simulink model "FMS1"  (R2018b)
settings: configuration reference "fms_config" (kept outside this file)
values from neighbouring files (symbols this model uses):
  FMS_EXPORT = Simulink.Parameter(FMS_EXPORT_VALUE)    [fms_model_init.m]
  FMS_PARAM = Simulink.Parameter(FMS_PARAM_VALUE)    [fms_model_init.m]
undefined symbols (not defined in the file or in its folder): actuator_cmd, ax_cmd, ay_cmd, az_cmd, cmd_mask, ControlMode, ctrl_mode, DiscIntNeverNeededParam, FMS_Cmd, FMS_CONST, home, mode, p_cmd, phi_cmd, PilotMode, psi_rate_cmd, q_cmd, r_cmd, reset, state, status, theta_cmd, throttle_cmd, timestamp, u_cmd, v_cmd, VehicleState, VehicleStatus, w_cmd, wp_consume, wp_current
libraries: simulink x119, FMT_Model_Lib x56, hdlsllib x13
(part 6 of 7)

== system FMS1/FMS Commander/Commander/Arm/Auto/Mission/Mission_SubSystem/Velocity Commander/Hold Position/Altitude Hold/Detect Movement ==
  FMS_In : Inport
  Abs : Abs
  Bus Selector : BusSelector  OutputSignals=INS_Out.vd
  Constant : Constant  Value=0  OutDataTypeStr=Inherit: Inherit via back propagation
  Motion Status : Stateflow chart  TreatAsAtomicUnit=on
  motion_state : Outport
  wires:
  FMS_In/1 -> Bus Selector/1
  Motion Status/1(state) -> motion_state/1
  Constant/1 -> Motion Status/1(motion_req)
  Abs/1 -> Motion Status/2(speed)
  Bus Selector/1 -> Abs/1  "<vd>"

== system FMS1/FMS Commander/Commander/Arm/Auto/Mission/Mission_SubSystem/Velocity Commander/Hold Position/Position Hold/Controller ==
  motion_state : Inport
  In Bus Element : Inport  Port=2  PortName=FMS_In
  In Bus Element1 : Inport  Port=2  PortName=FMS_In
  Brake Control : Subsystem  TreatAsAtomicUnit=on
  Hold Control : Subsystem  TreatAsAtomicUnit=on
  Merge : Merge  Inputs=3
  Move Control : Subsystem  TreatAsAtomicUnit=on
  Saturation1 : Saturate  UpperLimit=FMS_PARAM.VEL_XY_LIM  LowerLimit=-FMS_PARAM.VEL_XY_LIM
  Switch Case : SwitchCase  CaseConditions={MotionState.Hold, MotionState.Brake, MotionState.Move}  ShowDefaultCase=off
  uv_cmd_mPs : Outport
  wires:
  Move Control/1(uv_cmd_mPs) -> Merge/3
  Brake Control/1(uv_cmd_mPs) -> Merge/2
  Hold Control/1(uv_cmd_mPs) -> Merge/1
  In Bus Element/1 -> Hold Control/1(FMS_In)
  Switch Case/3 -> Move Control/Action
  Switch Case/2 -> Brake Control/Action
  Switch Case/1 -> Hold Control/Action
  motion_state/1 -> Switch Case/1
  Saturation1/1 -> uv_cmd_mPs/1
  Merge/1 -> Saturation1/1
  In Bus Element1/1 -> Move Control/1(FMS_In)

== system FMS1/FMS Commander/Commander/Arm/Auto/Mission/Mission_SubSystem/Velocity Commander/Hold Position/Position Hold/Detect Movement ==
  FMS_In : Inport
  Add : Sum
  Bus Selector1 : BusSelector  OutputSignals=INS_Out.vn,INS_Out.ve
  Constant : Constant  Value=0  OutDataTypeStr=Inherit: Inherit via back propagation
  Motion State : Stateflow chart  TreatAsAtomicUnit=on
  Sqrt : Sqrt  SaturateOnIntegerOverflow=on
  Square : Math  Operator=square  SaturateOnIntegerOverflow=on
  Square1 : Math  Operator=square  SaturateOnIntegerOverflow=on
  motion_state : Outport
  wires:
  FMS_In/1 -> Bus Selector1/1
  Add/1 -> Sqrt/1
  Square1/1 -> Add/2
  Square/1 -> Add/1
  Motion State/1(state) -> motion_state/1  "pos_ms"
  Sqrt/1 -> Motion State/2(speed)
  Bus Selector1/1 -> Square/1  "<vn>"
  Bus Selector1/2 -> Square1/1  "<ve>"
  Constant/1 -> Motion State/1(motion_req)

== system FMS1/FMS Commander/Commander/Arm/SubMode/Hold/Altitude Hold/Controller/Move Control/TD1/fhan  ==
  v1 : Inport
  v2 : Inport  Port=2
  Abs : Abs
  Add{,1..3,5..6} (6 alike) : Sum  OutDataTypeStr=Inherit: Same as first input
  Add4 : Sum  Inputs=-++
  Divide : Product  Inputs=*/
  Gain : Gain  Gain=8
  Gain1 : Gain  Gain=0.5  OutDataTypeStr=Inherit: Same as input
  Gain2 : Gain  Gain=0.5  OutDataTypeStr=Inherit: Same as input
  Gain3 : Gain  Gain=0.5  OutDataTypeStr=Inherit: Same as input
  Gain4 : Gain  Gain=-1  OutDataTypeStr=Inherit: Same as input
  Multiply{,1..3} (4 alike) : Product  OutDataTypeStr=Inherit: Same as first input
  Multiply4 : Product  OutDataTypeStr=single
  Multiply5 : Product  Inputs=3
  Multiply6 : Product  OutDataTypeStr=single
  Sign{,1..6} (7 alike) : Signum
  Sqrt : Sqrt  SaturateOnIntegerOverflow=on
  Square : Math  Operator=square  SaturateOnIntegerOverflow=on
  Subtract{,1..5} (6 alike) : Sum  Inputs=+-  OutDataTypeStr=Inherit: Same as first input
  Subtract6 : Sum  Inputs=-+  OutDataTypeStr=Inherit: Same as first input
  const : Constant  Value=r0  OutDataTypeStr=single
  const1 : Constant  Value=h0  OutDataTypeStr=single
  fhan : Outport
  wires:
  Sign1/1 -> Subtract2/1
  Multiply2/1 -> Sqrt/1
  Square/1 -> Multiply/2
  Gain1/1 -> Multiply3/2
  Multiply6/1 -> Subtract6/1
  Multiply/1 -> Multiply2/2, Add1/1, Add3/2, Subtract1/2, Add6/2, Subtract3/2, Divide/2, Subtract/2  "d"
  Add6/1 -> Sign3/1
  Sign3/1 -> Subtract4/1
  Sign6/1 -> Multiply6/1
  Multiply5/1 -> Subtract6/2
  Gain4/1 -> Multiply5/1
  Subtract4/1 -> Gain3/1
  Add2/1 -> Add5/1, Add4/1  "a2"
  Subtract2/1 -> Gain2/1
  Add/1 -> Abs/1, Sign/1, Add4/2, Add3/1, Subtract1/1  "y"
  Multiply1/1 -> Add/2, Add2/2, Add4/3  "a0"
  Add5/1 -> Add6/1, Subtract3/1, Divide/1, Sign5/1, Sign6/1  "a"
  const1/1 -> Square/1, Multiply1/2
  Multiply4/1 -> Add5/2
  Subtract5/1 -> Multiply5/2
  Add3/1 -> Sign1/1
  const/1 -> Multiply/1, Gain4/1, Multiply6/2
  Gain/1 -> Add1/2
  Multiply3/1 -> Add2/1
  Divide/1 -> Subtract5/1
  Subtract1/1 -> Sign2/1
  Add1/1 -> Multiply2/1
  Subtract3/1 -> Sign4/1
  Sqrt/1 -> Subtract/1  "a1"
  Sign5/1 -> Subtract5/2
  Add4/1 -> Multiply4/1
  Abs/1 -> Gain/1
  Sign4/1 -> Subtract4/2
  Sign2/1 -> Subtract2/2
  Subtract6/1 -> fhan/1
  Subtract/1 -> Gain1/1
  Gain3/1 -> Multiply5/3  "sa"
  v2/1 -> Multiply1/1
  Gain2/1 -> Multiply4/2  "sy"
  Sign/1 -> Multiply3/1
  v1/1 -> Add/1

== system FMS1/FMS Commander/Commander/Arm/SubMode/Hold/Heading Hold/Controller/Move Control/TD/fhan  ==
  v1 : Inport
  v2 : Inport  Port=2
  Abs : Abs
  Add{,1..3,5..6} (6 alike) : Sum  OutDataTypeStr=Inherit: Same as first input
  Add4 : Sum  Inputs=-++
  Divide : Product  Inputs=*/
  Gain : Gain  Gain=8
  Gain1 : Gain  Gain=0.5  OutDataTypeStr=Inherit: Same as input
  Gain2 : Gain  Gain=0.5  OutDataTypeStr=Inherit: Same as input
  Gain3 : Gain  Gain=0.5  OutDataTypeStr=Inherit: Same as input
  Gain4 : Gain  Gain=-1  OutDataTypeStr=Inherit: Same as input
  Multiply{,1..3} (4 alike) : Product  OutDataTypeStr=Inherit: Same as first input
  Multiply4 : Product  OutDataTypeStr=single
  Multiply5 : Product  Inputs=3
  Multiply6 : Product  OutDataTypeStr=single
  Sign{,1..6} (7 alike) : Signum
  Sqrt : Sqrt  SaturateOnIntegerOverflow=on
  Square : Math  Operator=square  SaturateOnIntegerOverflow=on
  Subtract{,1..5} (6 alike) : Sum  Inputs=+-  OutDataTypeStr=Inherit: Same as first input
  Subtract6 : Sum  Inputs=-+  OutDataTypeStr=Inherit: Same as first input
  const : Constant  Value=r0  OutDataTypeStr=single
  const1 : Constant  Value=h0  OutDataTypeStr=single
  fhan : Outport
  wires:
  v1/1 -> Add/1
  Sign/1 -> Multiply3/1
  Gain2/1 -> Multiply4/2  "sy"
  v2/1 -> Multiply1/1
  Gain3/1 -> Multiply5/3  "sa"
  Subtract/1 -> Gain1/1
  Subtract6/1 -> fhan/1
  Sign2/1 -> Subtract2/2
  Sign4/1 -> Subtract4/2
  Abs/1 -> Gain/1
  Add4/1 -> Multiply4/1
  Sign5/1 -> Subtract5/2
  Sqrt/1 -> Subtract/1  "a1"
  Subtract3/1 -> Sign4/1
  Add1/1 -> Multiply2/1
  Subtract1/1 -> Sign2/1
  Divide/1 -> Subtract5/1
  Multiply3/1 -> Add2/1
  Gain/1 -> Add1/2
  const/1 -> Multiply6/2, Gain4/1, Multiply/1
  Add3/1 -> Sign1/1
  Subtract5/1 -> Multiply5/2
  Multiply4/1 -> Add5/2
  const1/1 -> Multiply1/2, Square/1
  Add5/1 -> Sign6/1, Sign5/1, Divide/1, Subtract3/1, Add6/1  "a"
  Multiply1/1 -> Add4/3, Add2/2, Add/2  "a0"
  Add/1 -> Subtract1/1, Add3/1, Add4/2, Sign/1, Abs/1  "y"
  Subtract2/1 -> Gain2/1
  Add2/1 -> Add4/1, Add5/1  "a2"
  Subtract4/1 -> Gain3/1
  Gain4/1 -> Multiply5/1
  Multiply5/1 -> Subtract6/2
  Sign6/1 -> Multiply6/1
  Sign3/1 -> Subtract4/1
  Add6/1 -> Sign3/1
  Multiply/1 -> Subtract/2, Divide/2, Subtract3/2, Add6/2, Subtract1/2, Add3/2, Add1/1, Multiply2/2  "d"
  Multiply6/1 -> Subtract6/1
  Gain1/1 -> Multiply3/2
  Square/1 -> Multiply/2
  Multiply2/1 -> Sqrt/1
  Sign1/1 -> Subtract2/1

== system FMS1/FMS Commander/Commander/Arm/SubMode/Hold/Position Hold/Controller/Move Control/TD/fhan  ==
  v1 : Inport
  v2 : Inport  Port=2
  Abs : Abs
  Add{,1..3,5..6} (6 alike) : Sum  OutDataTypeStr=Inherit: Same as first input
  Add4 : Sum  Inputs=-++
  Divide : Product  Inputs=*/
  Gain : Gain  Gain=8
  Gain1 : Gain  Gain=0.5  OutDataTypeStr=Inherit: Same as input
  Gain2 : Gain  Gain=0.5  OutDataTypeStr=Inherit: Same as input
  Gain3 : Gain  Gain=0.5  OutDataTypeStr=Inherit: Same as input
  Gain4 : Gain  Gain=-1  OutDataTypeStr=Inherit: Same as input
  Multiply{,1..3} (4 alike) : Product  OutDataTypeStr=Inherit: Same as first input
  Multiply4 : Product  OutDataTypeStr=single
  Multiply5 : Product  Inputs=3
  Multiply6 : Product  OutDataTypeStr=single
  Sign{,1..6} (7 alike) : Signum
  Sqrt : Sqrt  SaturateOnIntegerOverflow=on
  Square : Math  Operator=square  SaturateOnIntegerOverflow=on
  Subtract{,1..5} (6 alike) : Sum  Inputs=+-  OutDataTypeStr=Inherit: Same as first input
  Subtract6 : Sum  Inputs=-+  OutDataTypeStr=Inherit: Same as first input
  const : Constant  Value=r0  OutDataTypeStr=single
  const1 : Constant  Value=h0  OutDataTypeStr=single
  fhan : Outport
  wires:
  v1/1 -> Add/1
  Sign/1 -> Multiply3/1
  Gain2/1 -> Multiply4/2  "sy"
  v2/1 -> Multiply1/1
  Gain3/1 -> Multiply5/3  "sa"
  Subtract/1 -> Gain1/1
  Subtract6/1 -> fhan/1
  Sign2/1 -> Subtract2/2
  Sign4/1 -> Subtract4/2
  Abs/1 -> Gain/1
  Add4/1 -> Multiply4/1
  Sign5/1 -> Subtract5/2
  Sqrt/1 -> Subtract/1  "a1"
  Subtract3/1 -> Sign4/1
  Add1/1 -> Multiply2/1
  Subtract1/1 -> Sign2/1
  Divide/1 -> Subtract5/1
  Multiply3/1 -> Add2/1
  Gain/1 -> Add1/2
  const/1 -> Multiply6/2, Gain4/1, Multiply/1
  Add3/1 -> Sign1/1
  Subtract5/1 -> Multiply5/2
  Multiply4/1 -> Add5/2
  const1/1 -> Multiply1/2, Square/1
  Add5/1 -> Sign6/1, Sign5/1, Divide/1, Subtract3/1, Add6/1  "a"
  Multiply1/1 -> Add4/3, Add2/2, Add/2  "a0"
  Add/1 -> Subtract1/1, Add3/1, Add4/2, Sign/1, Abs/1  "y"
  Subtract2/1 -> Gain2/1
  Add2/1 -> Add4/1, Add5/1  "a2"
  Subtract4/1 -> Gain3/1
  Gain4/1 -> Multiply5/1
  Multiply5/1 -> Subtract6/2
  Sign6/1 -> Multiply6/1
  Sign3/1 -> Subtract4/1
  Add6/1 -> Sign3/1
  Multiply/1 -> Subtract/2, Divide/2, Subtract3/2, Add6/2, Subtract1/2, Add3/2, Add1/1, Multiply2/2  "d"
  Multiply6/1 -> Subtract6/1
  Gain1/1 -> Multiply3/2
  Square/1 -> Multiply/2
  Multiply2/1 -> Sqrt/1
  Sign1/1 -> Subtract2/1

== system FMS1/FMS Commander/Commander/Arm/SubMode/Return/Velocity Commander1/Hold Position/Altitude Hold/Controller/Brake Control ==
  Action Port : ActionPort  InitializeStates=reset  ActionType=case
  Brake Speed : Constant  Value=0  VectorParams1D=off  OutDataTypeStr=single
  psi_rate_cmd_radPs : Outport
  wires:
  Brake Speed/1 -> psi_rate_cmd_radPs/1

== system FMS1/FMS Commander/Commander/Arm/SubMode/Return/Velocity Commander1/Hold Position/Altitude Hold/Controller/Hold Control ==
  FMS_In : Inport
  Action Port : ActionPort  InitializeStates=reset  ActionType=case
  Bus_Selection : Subsystem
  Delay : Delay  DelayLength=1  InitialConditionSource=Input port
      settings: InputPortMap=u0,p4
  Gain2 : Gain  Gain=FMS_PARAM.Z_P  OutDataTypeStr=single
  Sum : Sum  Inputs=-+|
  w_cmd_mPs : Outport
  wires:
  FMS_In/1 -> Bus_Selection/1(FMS_In)
  Delay/1 -> Sum/2, Delay/1  "z_cmd_R"
  Sum/1 -> Gain2/1  "z_err_R"
  Bus_Selection/1(z_R_m) -> Delay/2, Sum/1  "z_est_R"
  Gain2/1 -> w_cmd_mPs/1

== system FMS1/FMS Commander/Commander/Arm/SubMode/Return/Velocity Commander1/Hold Position/Altitude Hold/Controller/Move Control ==
  FMS_In : Inport
  Action Port : ActionPort  InitializeStates=reset  ActionType=case
  Bus Selector : BusSelector  OutputSignals=Pilot_Cmd.stick_throttle
  DeadZone : Subsystem  mask{th=FMS_PARAM.THROTTLE_DZ}
      mask prompts: th "Threshold"
      mask Display: disp('Dead Zone')
  Gain1 : Gain  Gain=-FMS_PARAM.VEL_Z_LIM  OutDataTypeStr=single
  TD1 : Subsystem
  w_cmd_mPs : Outport
  wires:
  TD1/1(v1) -> w_cmd_mPs/1
  FMS_In/1 -> Bus Selector/1
  Bus Selector/1 -> DeadZone/1(u)  "<stick_throttle>"
  DeadZone/1(y) -> Gain1/1
  Gain1/1 -> TD1/1(v)

== system FMS1/FMS Commander/Commander/Arm/SubMode/Return/Velocity Commander1/Hold Position/Position Hold/Controller/Brake Control ==
  Action Port : ActionPort  InitializeStates=reset  ActionType=case
  Brake Speed : Constant  Value=[0;0]  VectorParams1D=off  OutDataTypeStr=single
  uv_cmd_mPs : Outport
  wires:
  Brake Speed/1 -> uv_cmd_mPs/1

== system FMS1/FMS Commander/Commander/Arm/SubMode/Return/Velocity Commander1/Hold Position/Position Hold/Controller/Hold Control ==
  FMS_In : Inport
  Action Port : ActionPort  InitializeStates=reset  ActionType=case
  Bus Selector : BusSelector  OutputSignals=INS_Out.psi
  Bus_Selection : Subsystem
  Constant : Constant  Value=0  OutDataTypeStr=Inherit: Inherit via back propagation
  Delay : Delay  DelayLength=1  InitialConditionSource=Input port
      settings: InputPortMap=u0,p4
  Gain2 : Gain  Gain=FMS_PARAM.XY_P  OutDataTypeStr=single
  Multiply : Product  Multiplication=Matrix(*)
  Mux : Mux  Inputs=2
  Psi To DCM : FMT_Model_Lib/Transformation/Psi To DCM
      settings: SourceProductName=FMT Toolbox
  Selector : Selector  InputPortWidth=3  IndexOptions=Index vector (dialog)  Indices=[1 2]  OutputSizes=1
  Sum : Sum  Inputs=-+|
  uv_cmd_mPs : Outport
  wires:
  Bus Selector/1 -> Psi To DCM/1  "<psi>"
  Selector/1 -> Gain2/1
  Mux/1 -> Multiply/2
  Multiply/1 -> Selector/1
  Psi To DCM/1 -> Multiply/1  "M_CO"
  Constant/1 -> Mux/2
  FMS_In/1 -> Bus_Selection/1(FMS_In), Bus Selector/1
  Delay/1 -> Sum/2, Delay/1  "xy_cmd_R"
  Sum/1 -> Mux/1  "xy_err_R"
  Bus_Selection/1(xy_R_O_m) -> Delay/2, Sum/1  "xy_est_R"
  Gain2/1 -> uv_cmd_mPs/1

== system FMS1/FMS Commander/Commander/Arm/SubMode/Return/Velocity Commander1/Hold Position/Position Hold/Controller/Move Control ==
  FMS_In : Inport
  Action Port : ActionPort  InitializeStates=reset  ActionType=case
  Bus Selector : BusSelector  OutputSignals=Pilot_Cmd.stick_pitch,Pilot_Cmd.stick_roll
  DeadZone : Subsystem  mask{th=FMS_PARAM.PITCH_DZ}
      mask prompts: th "Threshold"
      mask Display: disp('Dead Zone')
  DeadZone1 : Subsystem  mask{th=FMS_PARAM.ROLL_DZ}
      mask prompts: th "Threshold"
      mask Display: disp('Dead Zone')
  Gain6 : Gain  Gain=FMS_PARAM.VEL_XY_LIM  OutDataTypeStr=single
  Mux1 : Mux  Inputs=2
  TD : Subsystem
  uv_cmd_mPs : Outport
  wires:
  Mux1/1 -> Gain6/1
  DeadZone1/1(y) -> Mux1/2
  Bus Selector/2 -> DeadZone1/1(u)  "<stick_roll>"
  TD/1(v1) -> uv_cmd_mPs/1
  FMS_In/1 -> Bus Selector/1
  Bus Selector/1 -> DeadZone/1(u)  "<stick_pitch>"
  DeadZone/1(y) -> Mux1/1
  Gain6/1 -> TD/1(v)

== system FMS1/FMS Commander/Commander/Arm/Auto/Mission/Mission_SubSystem/Velocity Commander/Hold Position/Altitude Hold/Controller/Brake Control ==
  Action Port : ActionPort  InitializeStates=reset  ActionType=case
  Brake Speed : Constant  Value=0  VectorParams1D=off  OutDataTypeStr=single
  psi_rate_cmd_radPs : Outport
  wires:
  Brake Speed/1 -> psi_rate_cmd_radPs/1

== system FMS1/FMS Commander/Commander/Arm/Auto/Mission/Mission_SubSystem/Velocity Commander/Hold Position/Altitude Hold/Controller/Hold Control ==
  FMS_In : Inport
  Action Port : ActionPort  InitializeStates=reset  ActionType=case
  Bus_Selection : Subsystem
  Delay : Delay  DelayLength=1  InitialConditionSource=Input port
      settings: InputPortMap=u0,p4
  Gain2 : Gain  Gain=FMS_PARAM.Z_P  OutDataTypeStr=single
  Sum : Sum  Inputs=-+|
  w_cmd_mPs : Outport
  wires:
  FMS_In/1 -> Bus_Selection/1(FMS_In)
  Delay/1 -> Sum/2, Delay/1  "z_cmd_R"
  Sum/1 -> Gain2/1  "z_err_R"
  Bus_Selection/1(z_R_m) -> Delay/2, Sum/1  "z_est_R"
  Gain2/1 -> w_cmd_mPs/1

== system FMS1/FMS Commander/Commander/Arm/Auto/Mission/Mission_SubSystem/Velocity Commander/Hold Position/Altitude Hold/Controller/Move Control ==
  FMS_In : Inport
  Action Port : ActionPort  InitializeStates=reset  ActionType=case
  Bus Selector : BusSelector  OutputSignals=Pilot_Cmd.stick_throttle
  DeadZone : Subsystem  mask{th=FMS_PARAM.THROTTLE_DZ}
      mask prompts: th "Threshold"
      mask Display: disp('Dead Zone')
  Gain1 : Gain  Gain=-FMS_PARAM.VEL_Z_LIM  OutDataTypeStr=single
  TD1 : Subsystem
  w_cmd_mPs : Outport
  wires:
  TD1/1(v1) -> w_cmd_mPs/1
  FMS_In/1 -> Bus Selector/1
  Bus Selector/1 -> DeadZone/1(u)  "<stick_throttle>"
  DeadZone/1(y) -> Gain1/1
  Gain1/1 -> TD1/1(v)

== system FMS1/FMS Commander/Commander/Arm/Auto/Mission/Mission_SubSystem/Velocity Commander/Hold Position/Position Hold/Controller/Brake Control ==
  Action Port : ActionPort  InitializeStates=reset  ActionType=case
  Brake Speed : Constant  Value=[0;0]  VectorParams1D=off  OutDataTypeStr=single
  uv_cmd_mPs : Outport
  wires:
  Brake Speed/1 -> uv_cmd_mPs/1

== system FMS1/FMS Commander/Commander/Arm/Auto/Mission/Mission_SubSystem/Velocity Commander/Hold Position/Position Hold/Controller/Hold Control ==
  FMS_In : Inport
  Action Port : ActionPort  InitializeStates=reset  ActionType=case
  Bus Selector : BusSelector  OutputSignals=INS_Out.psi
  Bus_Selection : Subsystem
  Constant : Constant  Value=0  OutDataTypeStr=Inherit: Inherit via back propagation
  Delay : Delay  DelayLength=1  InitialConditionSource=Input port
      settings: InputPortMap=u0,p4
  Gain2 : Gain  Gain=FMS_PARAM.XY_P  OutDataTypeStr=single
  Multiply : Product  Multiplication=Matrix(*)
  Mux : Mux  Inputs=2
  Psi To DCM : FMT_Model_Lib/Transformation/Psi To DCM
      settings: SourceProductName=FMT Toolbox
  Selector : Selector  InputPortWidth=3  IndexOptions=Index vector (dialog)  Indices=[1 2]  OutputSizes=1
  Sum : Sum  Inputs=-+|
  uv_cmd_mPs : Outport
  wires:
  Bus Selector/1 -> Psi To DCM/1  "<psi>"
  Selector/1 -> Gain2/1
  Mux/1 -> Multiply/2
  Multiply/1 -> Selector/1
  Psi To DCM/1 -> Multiply/1  "M_CO"
  Constant/1 -> Mux/2
  FMS_In/1 -> Bus_Selection/1(FMS_In), Bus Selector/1
  Delay/1 -> Sum/2, Delay/1  "xy_cmd_R"
  Sum/1 -> Mux/1  "xy_err_R"
  Bus_Selection/1(xy_R_O_m) -> Delay/2, Sum/1  "xy_est_R"
  Gain2/1 -> uv_cmd_mPs/1

== system FMS1/FMS Commander/Commander/Arm/Auto/Mission/Mission_SubSystem/Velocity Commander/Hold Position/Position Hold/Controller/Move Control ==
  FMS_In : Inport
  Action Port : ActionPort  InitializeStates=reset  ActionType=case
  Bus Selector : BusSelector  OutputSignals=Pilot_Cmd.stick_pitch,Pilot_Cmd.stick_roll
  DeadZone : Subsystem  mask{th=FMS_PARAM.PITCH_DZ}
      mask prompts: th "Threshold"
      mask Display: disp('Dead Zone')
  DeadZone1 : Subsystem  mask{th=FMS_PARAM.ROLL_DZ}
      mask prompts: th "Threshold"
      mask Display: disp('Dead Zone')
  Gain6 : Gain  Gain=FMS_PARAM.VEL_XY_LIM  OutDataTypeStr=single
  Mux1 : Mux  Inputs=2
  TD : Subsystem
  uv_cmd_mPs : Outport
  wires:
  Mux1/1 -> Gain6/1
  DeadZone1/1(y) -> Mux1/2
  Bus Selector/2 -> DeadZone1/1(u)  "<stick_roll>"
  TD/1(v1) -> uv_cmd_mPs/1
  FMS_In/1 -> Bus Selector/1
  Bus Selector/1 -> DeadZone/1(u)  "<stick_pitch>"
  DeadZone/1(y) -> Mux1/1
  Gain6/1 -> TD/1(v)

== system FMS1/FMS Commander/Commander/Arm/SubMode/Return/Velocity Commander1/Hold Position/Altitude Hold/Controller/Hold Control/Bus_Selection ==
  FMS_In : Inport
  Bus Selector2 : BusSelector  OutputSignals=INS_Out.h_R
  Gain : Gain  Gain=-1
  z_R_m : Outport
  wires:
  Gain/1 -> z_R_m/1
  Bus Selector2/1 -> Gain/1  "<h_R>"
  FMS_In/1 -> Bus Selector2/1

== system FMS1/FMS Commander/Commander/Arm/SubMode/Return/Velocity Commander1/Hold Position/Altitude Hold/Controller/Move Control/DeadZone ==
  u : Inport
  Dead Zone : DeadZone  LowerValue=-th  UpperValue=th  SaturateOnIntegerOverflow=on
  Gain : Gain  Gain=1/(1-th)
  y : Outport
  wires:
  Gain/1 -> y/1
  Dead Zone/1 -> Gain/1
  u/1 -> Dead Zone/1

== system FMS1/FMS Commander/Commander/Arm/SubMode/Return/Velocity Commander1/Hold Position/Altitude Hold/Controller/Move Control/TD1 ==
  v : Inport
  Integrator : DiscreteIntegrator  SampleTime=-1  ICPrevOutput=DiscIntNeverNeededParam  ICPrevScaledInput=DiscIntNeverNeededParam
  Integrator1 : DiscreteIntegrator  SampleTime=-1  ICPrevOutput=DiscIntNeverNeededParam  ICPrevScaledInput=DiscIntNeverNeededParam
  Subtract : Sum  Inputs=+-
  "fhan " : Subsystem  mask{r0=8*9.806, h0=0.05}
      mask DialogControl ParameterGroupVar Prompt: fhan(v1,v2,r0,h0)
  v1 : Outport
  wires:
  Integrator1/1 -> v1/1, Subtract/1
  v/1 -> Subtract/2
  Integrator/1 -> "fhan "/2(v2), Integrator1/1  "v2"
  Subtract/1 -> "fhan "/1(v1)
  "fhan "/1(fhan) -> Integrator/1

== system FMS1/FMS Commander/Commander/Arm/SubMode/Return/Velocity Commander1/Hold Position/Position Hold/Controller/Hold Control/Bus_Selection ==
  FMS_In : Inport
  Bus Selector2 : BusSelector  OutputSignals=INS_Out.x_R,INS_Out.y_R
  Mux : Mux  Inputs=2
  xy_R_O_m : Outport
  wires:
  Bus Selector2/2 -> Mux/2  "<y_R>"
  Mux/1 -> xy_R_O_m/1
  Bus Selector2/1 -> Mux/1  "<x_R>"
  FMS_In/1 -> Bus Selector2/1

== system FMS1/FMS Commander/Commander/Arm/SubMode/Return/Velocity Commander1/Hold Position/Position Hold/Controller/Move Control/DeadZone ==
  u : Inport
  Dead Zone : DeadZone  LowerValue=-th  UpperValue=th  SaturateOnIntegerOverflow=on
  Gain : Gain  Gain=1/(1-th)
  y : Outport
  wires:
  Gain/1 -> y/1
  Dead Zone/1 -> Gain/1
  u/1 -> Dead Zone/1

== system FMS1/FMS Commander/Commander/Arm/SubMode/Return/Velocity Commander1/Hold Position/Position Hold/Controller/Move Control/DeadZone1 ==
  u : Inport
  Dead Zone : DeadZone  LowerValue=-th  UpperValue=th  SaturateOnIntegerOverflow=on
  Gain : Gain  Gain=1/(1-th)
  y : Outport
  wires:
  u/1 -> Dead Zone/1
  Dead Zone/1 -> Gain/1
  Gain/1 -> y/1

== system FMS1/FMS Commander/Commander/Arm/SubMode/Return/Velocity Commander1/Hold Position/Position Hold/Controller/Move Control/TD ==
  v : Inport
  Integrator : DiscreteIntegrator  SampleTime=-1  ICPrevOutput=DiscIntNeverNeededParam  ICPrevScaledInput=DiscIntNeverNeededParam
  Integrator1 : DiscreteIntegrator  SampleTime=-1  ICPrevOutput=DiscIntNeverNeededParam  ICPrevScaledInput=DiscIntNeverNeededParam
  Subtract : Sum  Inputs=+-
  "fhan " : Subsystem  mask{r0=6*9.806, h0=0.05}
      mask DialogControl ParameterGroupVar Prompt: fhan(v1,v2,r0,h0)
  v1 : Outport
  wires:
  "fhan "/1(fhan) -> Integrator/1
  Subtract/1 -> "fhan "/1(v1)
  Integrator/1 -> Integrator1/1, "fhan "/2(v2)  "v2"
  v/1 -> Subtract/2
  Integrator1/1 -> Subtract/1, v1/1

== system FMS1/FMS Commander/Commander/Arm/Auto/Mission/Mission_SubSystem/Velocity Commander/Hold Position/Altitude Hold/Controller/Hold Control/Bus_Selection ==
  FMS_In : Inport
  Bus Selector2 : BusSelector  OutputSignals=INS_Out.h_R
  Gain : Gain  Gain=-1
  z_R_m : Outport
  wires:
  Gain/1 -> z_R_m/1
  Bus Selector2/1 -> Gain/1  "<h_R>"
  FMS_In/1 -> Bus Selector2/1

== system FMS1/FMS Commander/Commander/Arm/Auto/Mission/Mission_SubSystem/Velocity Commander/Hold Position/Altitude Hold/Controller/Move Control/DeadZone ==
  u : Inport
  Dead Zone : DeadZone  LowerValue=-th  UpperValue=th  SaturateOnIntegerOverflow=on
  Gain : Gain  Gain=1/(1-th)
  y : Outport
  wires:
  Gain/1 -> y/1
  Dead Zone/1 -> Gain/1
  u/1 -> Dead Zone/1

== system FMS1/FMS Commander/Commander/Arm/Auto/Mission/Mission_SubSystem/Velocity Commander/Hold Position/Altitude Hold/Controller/Move Control/TD1 ==
  v : Inport
  Integrator : DiscreteIntegrator  SampleTime=-1  ICPrevOutput=DiscIntNeverNeededParam  ICPrevScaledInput=DiscIntNeverNeededParam
  Integrator1 : DiscreteIntegrator  SampleTime=-1  ICPrevOutput=DiscIntNeverNeededParam  ICPrevScaledInput=DiscIntNeverNeededParam
  Subtract : Sum  Inputs=+-
  "fhan " : Subsystem  mask{r0=8*9.806, h0=0.05}
      mask DialogControl ParameterGroupVar Prompt: fhan(v1,v2,r0,h0)
  v1 : Outport
  wires:
  Integrator1/1 -> v1/1, Subtract/1
  v/1 -> Subtract/2
  Integrator/1 -> "fhan "/2(v2), Integrator1/1  "v2"
  Subtract/1 -> "fhan "/1(v1)
  "fhan "/1(fhan) -> Integrator/1

== system FMS1/FMS Commander/Commander/Arm/Auto/Mission/Mission_SubSystem/Velocity Commander/Hold Position/Position Hold/Controller/Hold Control/Bus_Selection ==
  FMS_In : Inport
  Bus Selector2 : BusSelector  OutputSignals=INS_Out.x_R,INS_Out.y_R
  Mux : Mux  Inputs=2
  xy_R_O_m : Outport
  wires:
  Bus Selector2/2 -> Mux/2  "<y_R>"
  Mux/1 -> xy_R_O_m/1
  Bus Selector2/1 -> Mux/1  "<x_R>"
  FMS_In/1 -> Bus Selector2/1

== system FMS1/FMS Commander/Commander/Arm/Auto/Mission/Mission_SubSystem/Velocity Commander/Hold Position/Position Hold/Controller/Move Control/DeadZone ==
  u : Inport
  Dead Zone : DeadZone  LowerValue=-th  UpperValue=th  SaturateOnIntegerOverflow=on
  Gain : Gain  Gain=1/(1-th)
  y : Outport
  wires:
  Gain/1 -> y/1
  Dead Zone/1 -> Gain/1
  u/1 -> Dead Zone/1

== system FMS1/FMS Commander/Commander/Arm/Auto/Mission/Mission_SubSystem/Velocity Commander/Hold Position/Position Hold/Controller/Move Control/DeadZone1 ==
  u : Inport
  Dead Zone : DeadZone  LowerValue=-th  UpperValue=th  SaturateOnIntegerOverflow=on
  Gain : Gain  Gain=1/(1-th)
  y : Outport
  wires:
  u/1 -> Dead Zone/1
  Dead Zone/1 -> Gain/1
  Gain/1 -> y/1

== system FMS1/FMS Commander/Commander/Arm/Auto/Mission/Mission_SubSystem/Velocity Commander/Hold Position/Position Hold/Controller/Move Control/TD ==
  v : Inport
  Integrator : DiscreteIntegrator  SampleTime=-1  ICPrevOutput=DiscIntNeverNeededParam  ICPrevScaledInput=DiscIntNeverNeededParam
  Integrator1 : DiscreteIntegrator  SampleTime=-1  ICPrevOutput=DiscIntNeverNeededParam  ICPrevScaledInput=DiscIntNeverNeededParam
  Subtract : Sum  Inputs=+-
  "fhan " : Subsystem  mask{r0=6*9.806, h0=0.05}
      mask DialogControl ParameterGroupVar Prompt: fhan(v1,v2,r0,h0)
  v1 : Outport
  wires:
  "fhan "/1(fhan) -> Integrator/1
  Subtract/1 -> "fhan "/1(v1)
  Integrator/1 -> Integrator1/1, "fhan "/2(v2)  "v2"
  v/1 -> Subtract/2
  Integrator1/1 -> Subtract/1, v1/1

== system FMS1/FMS Commander/Commander/Arm/SubMode/Return/Velocity Commander1/Hold Position/Altitude Hold/Controller/Move Control/TD1/fhan  ==
  v1 : Inport
  v2 : Inport  Port=2
  Abs : Abs
  Add{,1..3,5..6} (6 alike) : Sum  OutDataTypeStr=Inherit: Same as first input
  Add4 : Sum  Inputs=-++
  Divide : Product  Inputs=*/
  Gain : Gain  Gain=8
  Gain1 : Gain  Gain=0.5  OutDataTypeStr=Inherit: Same as input
  Gain2 : Gain  Gain=0.5  OutDataTypeStr=Inherit: Same as input
  Gain3 : Gain  Gain=0.5  OutDataTypeStr=Inherit: Same as input
  Gain4 : Gain  Gain=-1  OutDataTypeStr=Inherit: Same as input
  Multiply{,1..3} (4 alike) : Product  OutDataTypeStr=Inherit: Same as first input
  Multiply4 : Product  OutDataTypeStr=single
  Multiply5 : Product  Inputs=3
  Multiply6 : Product  OutDataTypeStr=single
  Sign{,1..6} (7 alike) : Signum
  Sqrt : Sqrt  SaturateOnIntegerOverflow=on
  Square : Math  Operator=square  SaturateOnIntegerOverflow=on
  Subtract{,1..5} (6 alike) : Sum  Inputs=+-  OutDataTypeStr=Inherit: Same as first input
  Subtract6 : Sum  Inputs=-+  OutDataTypeStr=Inherit: Same as first input
  const : Constant  Value=r0  OutDataTypeStr=single
  const1 : Constant  Value=h0  OutDataTypeStr=single
  fhan : Outport
  wires:
  Sign1/1 -> Subtract2/1
  Multiply2/1 -> Sqrt/1
  Square/1 -> Multiply/2
  Gain1/1 -> Multiply3/2
  Multiply6/1 -> Subtract6/1
  Multiply/1 -> Multiply2/2, Add1/1, Add3/2, Subtract1/2, Add6/2, Subtract3/2, Divide/2, Subtract/2  "d"
  Add6/1 -> Sign3/1
  Sign3/1 -> Subtract4/1
  Sign6/1 -> Multiply6/1
  Multiply5/1 -> Subtract6/2
  Gain4/1 -> Multiply5/1
  Subtract4/1 -> Gain3/1
  Add2/1 -> Add5/1, Add4/1  "a2"
  Subtract2/1 -> Gain2/1
  Add/1 -> Abs/1, Sign/1, Add4/2, Add3/1, Subtract1/1  "y"
  Multiply1/1 -> Add/2, Add2/2, Add4/3  "a0"
  Add5/1 -> Add6/1, Subtract3/1, Divide/1, Sign5/1, Sign6/1  "a"
  const1/1 -> Square/1, Multiply1/2
  Multiply4/1 -> Add5/2
  Subtract5/1 -> Multiply5/2
  Add3/1 -> Sign1/1
  const/1 -> Multiply/1, Gain4/1, Multiply6/2
  Gain/1 -> Add1/2
  Multiply3/1 -> Add2/1
  Divide/1 -> Subtract5/1
  Subtract1/1 -> Sign2/1
  Add1/1 -> Multiply2/1
  Subtract3/1 -> Sign4/1
  Sqrt/1 -> Subtract/1  "a1"
  Sign5/1 -> Subtract5/2
  Add4/1 -> Multiply4/1
  Abs/1 -> Gain/1
  Sign4/1 -> Subtract4/2
  Sign2/1 -> Subtract2/2
  Subtract6/1 -> fhan/1
  Subtract/1 -> Gain1/1
  Gain3/1 -> Multiply5/3  "sa"
  v2/1 -> Multiply1/1
  Gain2/1 -> Multiply4/2  "sy"
  Sign/1 -> Multiply3/1
  v1/1 -> Add/1

== system FMS1/FMS Commander/Commander/Arm/SubMode/Return/Velocity Commander1/Hold Position/Position Hold/Controller/Move Control/TD/fhan  ==
  v1 : Inport
  v2 : Inport  Port=2
  Abs : Abs
  Add{,1..3,5..6} (6 alike) : Sum  OutDataTypeStr=Inherit: Same as first input
  Add4 : Sum  Inputs=-++
  Divide : Product  Inputs=*/
  Gain : Gain  Gain=8
  Gain1 : Gain  Gain=0.5  OutDataTypeStr=Inherit: Same as input
  Gain2 : Gain  Gain=0.5  OutDataTypeStr=Inherit: Same as input
  Gain3 : Gain  Gain=0.5  OutDataTypeStr=Inherit: Same as input
  Gain4 : Gain  Gain=-1  OutDataTypeStr=Inherit: Same as input
  Multiply{,1..3} (4 alike) : Product  OutDataTypeStr=Inherit: Same as first input
  Multiply4 : Product  OutDataTypeStr=single
  Multiply5 : Product  Inputs=3
  Multiply6 : Product  OutDataTypeStr=single
  Sign{,1..6} (7 alike) : Signum
  Sqrt : Sqrt  SaturateOnIntegerOverflow=on
  Square : Math  Operator=square  SaturateOnIntegerOverflow=on
  Subtract{,1..5} (6 alike) : Sum  Inputs=+-  OutDataTypeStr=Inherit: Same as first input
  Subtract6 : Sum  Inputs=-+  OutDataTypeStr=Inherit: Same as first input
  const : Constant  Value=r0  OutDataTypeStr=single
  const1 : Constant  Value=h0  OutDataTypeStr=single
  fhan : Outport
  wires:
  v1/1 -> Add/1
  Sign/1 -> Multiply3/1
  Gain2/1 -> Multiply4/2  "sy"
  v2/1 -> Multiply1/1
  Gain3/1 -> Multiply5/3  "sa"
  Subtract/1 -> Gain1/1
  Subtract6/1 -> fhan/1
  Sign2/1 -> Subtract2/2
  Sign4/1 -> Subtract4/2
  Abs/1 -> Gain/1
  Add4/1 -> Multiply4/1
  Sign5/1 -> Subtract5/2
  Sqrt/1 -> Subtract/1  "a1"
  Subtract3/1 -> Sign4/1
  Add1/1 -> Multiply2/1
  Subtract1/1 -> Sign2/1
  Divide/1 -> Subtract5/1
  Multiply3/1 -> Add2/1
  Gain/1 -> Add1/2
  const/1 -> Multiply6/2, Gain4/1, Multiply/1
  Add3/1 -> Sign1/1
  Subtract5/1 -> Multiply5/2
  Multiply4/1 -> Add5/2
  const1/1 -> Multiply1/2, Square/1
  Add5/1 -> Sign6/1, Sign5/1, Divide/1, Subtract3/1, Add6/1  "a"
  Multiply1/1 -> Add4/3, Add2/2, Add/2  "a0"
  Add/1 -> Subtract1/1, Add3/1, Add4/2, Sign/1, Abs/1  "y"
  Subtract2/1 -> Gain2/1
  Add2/1 -> Add4/1, Add5/1  "a2"
  Subtract4/1 -> Gain3/1
  Gain4/1 -> Multiply5/1
  Multiply5/1 -> Subtract6/2
  Sign6/1 -> Multiply6/1
  Sign3/1 -> Subtract4/1
  Add6/1 -> Sign3/1
  Multiply/1 -> Subtract/2, Divide/2, Subtract3/2, Add6/2, Subtract1/2, Add3/2, Add1/1, Multiply2/2  "d"
  Multiply6/1 -> Subtract6/1
  Gain1/1 -> Multiply3/2
  Square/1 -> Multiply/2
  Multiply2/1 -> Sqrt/1
  Sign1/1 -> Subtract2/1

== system FMS1/FMS Commander/Commander/Arm/Auto/Mission/Mission_SubSystem/Velocity Commander/Hold Position/Altitude Hold/Controller/Move Control/TD1/fhan  ==
  v1 : Inport
  v2 : Inport  Port=2
  Abs : Abs
  Add{,1..3,5..6} (6 alike) : Sum  OutDataTypeStr=Inherit: Same as first input
  Add4 : Sum  Inputs=-++
  Divide : Product  Inputs=*/
  Gain : Gain  Gain=8
  Gain1 : Gain  Gain=0.5  OutDataTypeStr=Inherit: Same as input
  Gain2 : Gain  Gain=0.5  OutDataTypeStr=Inherit: Same as input
  Gain3 : Gain  Gain=0.5  OutDataTypeStr=Inherit: Same as input
  Gain4 : Gain  Gain=-1  OutDataTypeStr=Inherit: Same as input
  Multiply{,1..3} (4 alike) : Product  OutDataTypeStr=Inherit: Same as first input
  Multiply4 : Product  OutDataTypeStr=single
  Multiply5 : Product  Inputs=3
  Multiply6 : Product  OutDataTypeStr=single
  Sign{,1..6} (7 alike) : Signum
  Sqrt : Sqrt  SaturateOnIntegerOverflow=on
  Square : Math  Operator=square  SaturateOnIntegerOverflow=on
  Subtract{,1..5} (6 alike) : Sum  Inputs=+-  OutDataTypeStr=Inherit: Same as first input
  Subtract6 : Sum  Inputs=-+  OutDataTypeStr=Inherit: Same as first input
  const : Constant  Value=r0  OutDataTypeStr=single
  const1 : Constant  Value=h0  OutDataTypeStr=single
  fhan : Outport
  wires:
  Sign1/1 -> Subtract2/1
  Multiply2/1 -> Sqrt/1
  Square/1 -> Multiply/2
  Gain1/1 -> Multiply3/2
  Multiply6/1 -> Subtract6/1
  Multiply/1 -> Multiply2/2, Add1/1, Add3/2, Subtract1/2, Add6/2, Subtract3/2, Divide/2, Subtract/2  "d"
  Add6/1 -> Sign3/1
  Sign3/1 -> Subtract4/1
  Sign6/1 -> Multiply6/1
  Multiply5/1 -> Subtract6/2
  Gain4/1 -> Multiply5/1
  Subtract4/1 -> Gain3/1
  Add2/1 -> Add5/1, Add4/1  "a2"
  Subtract2/1 -> Gain2/1
  Add/1 -> Abs/1, Sign/1, Add4/2, Add3/1, Subtract1/1  "y"
  Multiply1/1 -> Add/2, Add2/2, Add4/3  "a0"
  Add5/1 -> Add6/1, Subtract3/1, Divide/1, Sign5/1, Sign6/1  "a"
  const1/1 -> Square/1, Multiply1/2
  Multiply4/1 -> Add5/2
  Subtract5/1 -> Multiply5/2
  Add3/1 -> Sign1/1
  const/1 -> Multiply/1, Gain4/1, Multiply6/2
  Gain/1 -> Add1/2
  Multiply3/1 -> Add2/1
  Divide/1 -> Subtract5/1
  Subtract1/1 -> Sign2/1
  Add1/1 -> Multiply2/1
  Subtract3/1 -> Sign4/1
  Sqrt/1 -> Subtract/1  "a1"
  Sign5/1 -> Subtract5/2
  Add4/1 -> Multiply4/1
  Abs/1 -> Gain/1
  Sign4/1 -> Subtract4/2
  Sign2/1 -> Subtract2/2
  Subtract6/1 -> fhan/1
  Subtract/1 -> Gain1/1
  Gain3/1 -> Multiply5/3  "sa"
  v2/1 -> Multiply1/1
  Gain2/1 -> Multiply4/2  "sy"
  Sign/1 -> Multiply3/1
  v1/1 -> Add/1

== system FMS1/FMS Commander/Commander/Arm/Auto/Mission/Mission_SubSystem/Velocity Commander/Hold Position/Position Hold/Controller/Move Control/TD/fhan  ==
  v1 : Inport
  v2 : Inport  Port=2
  Abs : Abs
  Add{,1..3,5..6} (6 alike) : Sum  OutDataTypeStr=Inherit: Same as first input
  Add4 : Sum  Inputs=-++
  Divide : Product  Inputs=*/
  Gain : Gain  Gain=8
  Gain1 : Gain  Gain=0.5  OutDataTypeStr=Inherit: Same as input
  Gain2 : Gain  Gain=0.5  OutDataTypeStr=Inherit: Same as input
  Gain3 : Gain  Gain=0.5  OutDataTypeStr=Inherit: Same as input
  Gain4 : Gain  Gain=-1  OutDataTypeStr=Inherit: Same as input
  Multiply{,1..3} (4 alike) : Product  OutDataTypeStr=Inherit: Same as first input
  Multiply4 : Product  OutDataTypeStr=single
  Multiply5 : Product  Inputs=3
  Multiply6 : Product  OutDataTypeStr=single
  Sign{,1..6} (7 alike) : Signum
  Sqrt : Sqrt  SaturateOnIntegerOverflow=on
  Square : Math  Operator=square  SaturateOnIntegerOverflow=on
  Subtract{,1..5} (6 alike) : Sum  Inputs=+-  OutDataTypeStr=Inherit: Same as first input
  Subtract6 : Sum  Inputs=-+  OutDataTypeStr=Inherit: Same as first input
  const : Constant  Value=r0  OutDataTypeStr=single
  const1 : Constant  Value=h0  OutDataTypeStr=single
  fhan : Outport
  wires:
  v1/1 -> Add/1
  Sign/1 -> Multiply3/1
  Gain2/1 -> Multiply4/2  "sy"
  v2/1 -> Multiply1/1
  Gain3/1 -> Multiply5/3  "sa"
  Subtract/1 -> Gain1/1
  Subtract6/1 -> fhan/1
  Sign2/1 -> Subtract2/2
  Sign4/1 -> Subtract4/2
  Abs/1 -> Gain/1
  Add4/1 -> Multiply4/1
  Sign5/1 -> Subtract5/2
  Sqrt/1 -> Subtract/1  "a1"
  Subtract3/1 -> Sign4/1
  Add1/1 -> Multiply2/1
  Subtract1/1 -> Sign2/1
  Divide/1 -> Subtract5/1
  Multiply3/1 -> Add2/1
  Gain/1 -> Add1/2
  const/1 -> Multiply6/2, Gain4/1, Multiply/1
  Add3/1 -> Sign1/1
  Subtract5/1 -> Multiply5/2
  Multiply4/1 -> Add5/2
  const1/1 -> Multiply1/2, Square/1
  Add5/1 -> Sign6/1, Sign5/1, Divide/1, Subtract3/1, Add6/1  "a"
  Multiply1/1 -> Add4/3, Add2/2, Add/2  "a0"
  Add/1 -> Subtract1/1, Add3/1, Add4/2, Sign/1, Abs/1  "y"
  Subtract2/1 -> Gain2/1
  Add2/1 -> Add4/1, Add5/1  "a2"
  Subtract4/1 -> Gain3/1
  Gain4/1 -> Multiply5/1
  Multiply5/1 -> Subtract6/2
  Sign6/1 -> Multiply6/1
  Sign3/1 -> Subtract4/1
  Add6/1 -> Sign3/1
  Multiply/1 -> Subtract/2, Divide/2, Subtract3/2, Add6/2, Subtract1/2, Add3/2, Add1/1, Multiply2/2  "d"
  Multiply6/1 -> Subtract6/1
  Gain1/1 -> Multiply3/2
  Square/1 -> Multiply/2
  Multiply2/1 -> Sqrt/1
  Sign1/1 -> Subtract2/1

== stateflow chart FMS1/SafeMode ==
  state Other
  state Offboard
  state Mission
  state Position
  state Altitude
  state Stabilize
  state Acro
  state Manual
  (junction 21) -> Other
  Other -> (junction 68) : {target_mode = mode;}
  (junction 78) -> (junction 21) [order 2]
  (junction 68) -> (junction 80)
  (junction 78) -> Offboard [order 1] : [mode == PilotMode.Offboard]
  Offboard -> (junction 77)
  (junction 77) -> (junction 80) [order 1] : [bitget(flag, 3)&&bitget(flag, 5)&&bitget(flag, 7)&&bitget(flag, 8)]
      | {target_mode = PilotMode.Offboard;}
  (junction 1) -> (junction 78) [order 2]
  (junction 77) -> Position [order 2]
  (junction 80) -> (junction 48)
  (junction 1) -> Mission [order 1] : [mode == PilotMode.Mission]
  Mission -> (junction 16)
  (junction 16) -> (junction 48) [order 1] : [bitget(flag, 3)&&bitget(flag, 5)&&bitget(flag, 6)&&bitget(flag, 7)&&bitget(flag, 8)]
      | {target_mode = PilotMode.Mission;}
  (junction 16) -> Position [order 2]
  (junction 47) -> (junction 1) [order 2]
  (junction 48) -> (junction 51)
  (junction 47) -> Position [order 1] : [mode == PilotMode.Position]
  Position -> (junction 49)
  (junction 49) -> (junction 51) [order 1] : [bitget(flag, 3)&&bitget(flag, 5)&&bitget(flag, 7)&&bitget(flag, 8)]
      | {target_mode = PilotMode.Position;}
  (junction 55) -> (junction 47) [order 2]
  (junction 49) -> Altitude [order 2]
  (junction 51) -> (junction 2)
  (junction 55) -> Altitude [order 1] : [mode == PilotMode.Altitude]
  Altitude -> (junction 28)
  (junction 28) -> (junction 2) [order 1] : [bitget(flag, 3)&&bitget(flag, 8)]
      | {target_mode = PilotMode.Altitude;}
  (junction 24) -> (junction 55) [order 2]
  (junction 28) -> Stabilize [order 2]
  (junction 2) -> (junction 39)
  (junction 24) -> Stabilize [order 1] : [mode == PilotMode.Stabilize]
  Stabilize -> (junction 44)
  (junction 44) -> (junction 39) [order 1] : [bitget(flag, 3)]{target_mode = PilotMode.Stabilize;}
  (junction 35) -> (junction 24) [order 2]
  (junction 44) -> Acro [order 2]
  (junction 39) -> (junction 53)
  (junction 35) -> Acro [order 1] : [mode == PilotMode.Acro]
  Acro -> (junction 22)
  (junction 22) -> (junction 53) [order 1] : [bitget(flag, 3)]{target_mode = PilotMode.Acro;}
  (junction 10) -> (junction 35) [order 2]
  (junction 22) -> Manual [order 2]
  (junction 53) -> (junction 15)
  (default) -> (junction 10)
  (junction 10) -> Manual [order 1] : [mode == PilotMode.Manual]
  Manual -> (junction 15) : {target_mode = PilotMode.Manual;}
  (junction 41) -> (junction 10)
  (junction 15) -> (junction 40)
  (junction 40) -> (junction 41)
  data: target_mode output; mode input Enum: PilotMode; flag input uint32

== stateflow chart FMS1/FMS Commander/Commander/Arm/Auto/Mission/Mission_SubSystem/Velocity Commander/Hold Position/Altitude Hold/Detect Movement/Motion Status ==
  state Hold
    entry:
    state=MotionState.Hold;
  state Move
    entry:
    state=MotionState.Move;
  state Brake
    entry:
    state=MotionState.Brake;
  (default) -> Move
  Hold -> Move : [motion_req==1]
  Move -> Brake : [motion_req==0]
  Brake -> Move [order 2] : [motion_req==1]
  Brake -> Hold [order 1] : [speed<=0.15 || after(1.5, sec)]
  data: state output Enum: MotionState; motion_req input; speed input

== stateflow chart FMS1/FMS Commander/Commander/Arm/Auto/Mission/Mission_SubSystem/Velocity Commander/Hold Position/Position Hold/Detect Movement/Motion State ==
  state Hold
    entry:
    state=MotionState.Hold;
  state Move
    entry:
    state=MotionState.Move;
  state Brake
    entry:
    state=MotionState.Brake;
  (default) -> Move
  Hold -> Move : [motion_req==1]
  Move -> Brake : [motion_req==0]
  Brake -> Move [order 2] : [motion_req==1]
  Brake -> Hold [order 1] : [speed<=0.2 || after(2.5, sec)]
  data: state output Enum: MotionState; motion_req input; speed input

== matlab function FMS1/FMS Commander/Commander/Arm/Auto/Mission/Mission_SubSystem/Velocity Commander/L1 Reference WP/NearbyRefWP ==
  data: P output; P2 input; d output; P3 input; L1 input
% Find the reference waypoint when vehicle (P3) is close to target (P2)
%
% If the vehicle is close to target (distance(P2,P3) < L1), select P2 as
% reference waypoint and return the distance, otherwise return -1.
function [P,d] = NearbyRefWP(P2, P3, L1)

P3P2 = P2 - P3;
dis = sqrt(sum(P3P2.^2));

if dis <= L1
    d = dis;
    % select P2 as reference WP
    P = P2;
else
    d = single(-1);
    % unset WP
    P = single([0; 0]);
end

== matlab function FMS1/FMS Commander/Commander/Arm/Auto/Mission/Mission_SubSystem/Velocity Commander/L1 Reference WP/OutRegionRegWP ==
  data: P1 input; P output; P2 input; P3 input
% Find the reference waypoint when vehicle is out of L1 region near P1P2.
%
% There are three region defined:
%   Region 1: The project point of P3 is lied on left side of P1P2
%   Region 2: The project point of P3 is lied on right side of P1P2
%   Region 3: The project point of P3 is lied on the segment line 
%
%   For the case of region 3, we select the project point as the reference
%   wayspoint. For the case of region 1, we choose P1 as reference waypoint
%   and similarly for the case of region 2, we choose P3 as reference
%   waypoint.
function P = OutRegionRefWP(P1, P2, P3)
% segment line P1P2
P1P2 = P2 - P1;
% segment line P1P3
P1P3 = P3 - P1;

% Define C as the P3 project point on line P1P2.
% Hence, P1C = dot(P1P3, P1P2)/|P1P2| * (P1P2/|P1P2|) = u * P1P2
% where u = dot(P1P3, P1P2) / |P1P2|^2.
u = dot(P1P3, P1P2) / sum(P1P2.^2);

if u <= 0
    % region 1
    P = P1;
elseif u >= 1
    % region 2
    P = P2;
else
    % region 3. C = P1C + P1
    P = u * P1P2 + P1;
end

== matlab function FMS1/FMS Commander/Commander/Arm/Auto/Mission/Mission_SubSystem/Velocity Commander/L1 Reference WP/SearchL1RefWP ==
  data: P1 input; P output; P2 input; P3 input; L1 input; u output
% Find reference waypoint (L1RefWP) on the line segment P1P2 which has 
% L1 distance from vehicle position (P3).
%
% The idea is to calculate the intersection point of a circle with L1 radius
% with the line segment P1P2.
%
% Define P = P1 + u * (P2 - P1), where P is the intersection point.
% Goal is calculating the u, where the valid u is between [0, 1].
%
% Input:
%   P1: start point of segment line
%   P2: start point of segment line
%   P3: circle center point, also is known as the vehicle position
%   L1: the L1 distance
% Output:
%   P: L1 reference waypoint
%   u: scale factor (valid between 0 and 1), -1 means no intersection.
function [P, u] = SearchL1RefWP(P1, P2, P3, L1)

% P1 = (x1, y1), P2 = (x2, y2), P3 = (x3, y3)
x1 = P1(1);
y1 = P1(2);
x2 = P2(1);
y2 = P2(2);
x3 = P3(1);
y3 = P3(2);

% The P is on circle and line segment, which yields:
A = (x2 - x1)^2 + (y2 - y1)^2;
B = 2 * ((x2 - x1)*(x1 - x3) + (y2 - y1)*(y1 - y3));
C = x3^2 + y3^2 + x1^2 + y1^2 - 2*(x3*x1 + y3*y1) - L1^2;
% Check root existence confition if B^2 - 4*A*C >= 0
D = B^2 - 4*A*C;
u = single(-1);
P = single([0 0]);

if D > 0
    % D>0 means we have 2 difference roots, % root is valid only if u is in range of [0, 1]
    u1 = (-B + sqrt(D)) / (2*A);
    u2 = (-B - sqrt(D)) / (2*A);
    
    if (u1>=0 && u1<=1) && (u2>=0 && u2<=1)
        % have 2 valid roots, select the one which is closer to P2 (target point)
        if u1 > u2
            u = u1; 
        else
            u = u2;
        end
    elseif (u1>=0 && u1<=1)
        % only 1 root valid, select it
        u = u1;
    elseif (u2>=0 && u2<=1)
        % only 1 root valid, select it
        u = u2;
    else
        % no valid root, which means no intersection point founded.
        return;
    end
elseif D == 0
    % D=0 means only 1 single root
    u1 = -B / (2*A);
    if (u1>=0 && u1<=1)
        % valid root, select it
        u = u1;
    else
        % no valid root, which means no intersection point founded.
        return;
    end
else
    % no valid root, which means no intersection point founded.
    return;
end

% calculate the L1 reference waypoint (P) coordinate
P(1) = x1 + u*(x2 - x1);
P(2) = y1 + u*(y2 - y1);

== stateflow chart FMS1/FMS Commander/Commander/Arm/SubMode/Return/Velocity Commander1/Hold Position/Altitude Hold/Detect Movement/Motion Status ==
  state Hold
    entry:
    state=MotionState.Hold;
  state Move
    entry:
    state=MotionState.Move;
  state Brake
    entry:
    state=MotionState.Brake;
  (default) -> Move
  Hold -> Move : [motion_req==1]
  Move -> Brake : [motion_req==0]
  Brake -> Move [order 2] : [motion_req==1]
  Brake -> Hold [order 1] : [speed<=0.15 || after(1.5, sec)]
  data: state output Enum: MotionState; motion_req input; speed input
